simulink library "Cylinder_Lib"  (R2025a)
settings: Solver=ode45  StartTime=0.0  StopTime=10.0  RelTol=1e-3  EnableMultiTasking=on
undefined symbols (not defined in the file or in its folder): actuator_hs_b, actuator_hs_k
libraries: fl_lib x9, SimscapeFluids_lib x1
Description:
  | Copyright 2015-2025 The MathWorks, Inc.
settings Model: Creator=smiller  LastModifiedBy=smiller
settings SolverCC: AlgebraicLoopSolver=TrustRegion
settings DataIOCC: LimitDataPoints=on  SaveFormat=Array  ReturnWorkspaceOutputs=off
settings OptimizationCC: ReuseModelBlockBuffer=off  ExpressionDepthLimit=2147483647.0  LifeSpan=inf
settings DebuggingCC: UnderspecifiedInitializationDetection=Classic  MergeDetectMultiDrivingBlocksExec=none  SolverPrmCheckMsg=warning  UnconnectedInputMsg=warning  UnconnectedOutputMsg=warning  UnconnectedLineMsg=warning  AllowSymbolicDim=off  StateNameClashWarn=warning  PregeneratedLibrarySubsystemCodeDiagnostic=none  SFUnexpectedBacktrackingDiag=warning  SFNoUnconditionalDefaultTransitionDiag=warning  SFExecutionAtInitializationDiag=none  ArithmeticOperatorsInVariantConditions=warning
settings HardwareCC: ProdBitPerPointer=32.0  ProdBitPerSizeT=32.0  ProdBitPerPtrDiffT=32.0  ProdLargestAtomicFloat=None  ProdIntDivRoundTo=Undefined  ProdEndianess=Unspecified  ProdWordSize=32.0  ProdHWDeviceType=32-bit Generic
settings ModelReferenceCC: EnableRefExpFcnMdlSchedulingChecks=on  PropagateSignalLabelsOutOfModel=off
settings SFSimCC: SimUseLocalCustomCode=off  CustomCodeUndefinedFunction=UseInterfaceOnly
settings RTWCC: RTWUseLocalCustomCode=off  GPUComputeCapability=3.5  DLArmComputeVersion=19.05
settings CodeAppCC: StateflowObjectComments=on
settings GRTTargetCC: TargetLangStandard=C89/C90 (ANSI)
settings ConfigComp: CovMetricSettings=dw  CovSaveCumulativeToWorkspaceVar=on  CovSaveSingleToWorkspaceVar=on  CovExternalEMLEnable=off  CovSFcnEnable=off

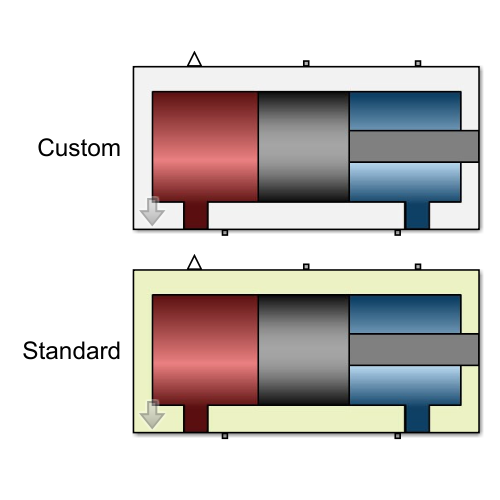
[thumbnail: Simulink's stored preview of the top-level diagram]
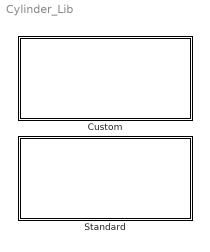
== system Cylinder_Lib ==
  Custom : Subsystem  VariantControl=Custom  mask(Double-Acting Hydraulic Actuator){A=5e-4, V=10e-5, PA=200, PB=0, T=200, hs_k=actuator_hs_k, hs_b=actuator_hs_b}
      mask prompts: A "Piston area (m^2)"; V "Chamber dead volume (m^3)"; PA "Chamber A initial pressure (bar)"; PB "Chamber B initial pressure (bar)"; T "Piston travel (mm)"; hs_k "Hardstop stiffness (N/m)"; hs_b "Hardstop damping (N/(m/s))"
      mask help: Models a double-acting hydraulic actuator using Simscape Foundation library components.
      mask Display: image('Double_Acting_Cylinder_Custom_IMAGE.jpg');
  Standard : Subsystem  VariantControl=Standard  mask(Double-Acting Hydraulic Actuator){A=5e-4, V=10e-5, PA=200, PB=0, T=200, hs_k=actuator_hs_k, hs_b=actuator_hs_b}
      mask prompts: A "Piston area (m^2)"; V "Chamber dead volume (m^3)"; PA "Chamber A initial pressure (bar)"; PB "Chamber B initial pressure (bar)"; T "Piston travel (mm)"; hs_k "Hardstop stiffness (N/m)"; hs_b "Hardstop damping (N/(m/s))"
      mask help: Models a double-acting hydraulic actuator using Simscape add-on library components.
      mask Display: image('Double_Acting_Cylinder_Standard_IMAGE.jpg');

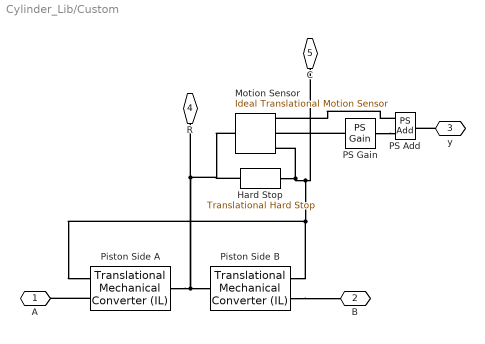
== system Cylinder_Lib/Custom ==
  " Motion Sensor" : fl_lib/Mechanical/Mechanical Sensors/Ideal Translational Motion Sensor  reference=foundation.enum.MeasurementReference.difference  acceleration_port=false  velocity_port=true  position_port=true  offset=Scissor_Lift_Param.Initial_Cyl_Ext mm
  Hard Stop : fl_lib/Mechanical/Translational Elements/Translational Hard Stop  upper_bnd=T/2 mm  lower_bnd=-T/2 mm  model=3  stiff_up=hs_k N/m  stiff_low=hs_k N/m  D_up=hs_b N/(m/s)  D_low=hs_b N/(m/s)  transition=0.1 mm  coeff_rest=0.7  v_tol=0.001 m/s  f_tol=0.001 N  v_specify=off  v_priority=High  v=0 m/s  v_nominal_specify=off  v_nominal_value=1  v_nominal_unit=m/s  f_specify=off  f_priority=High  f=0 N  f_nominal_specify=off  f_nominal_value=1  f_nominal_unit=N  x_specify=on  x_priority=High  x=0 m  x_nominal_specify=off  x_nominal_value=1  x_nominal_unit=m  M_specify=off  M_priority=None  M=0
  PS Add : fl_lib/Physical Signals/Functions/PS Add
  PS Gain : fl_lib/Physical Signals/Functions/PS Gain  gain=0.1 s
  Piston Side A : fl_lib/Isothermal Liquid/Elements/Translational Mechanical Converter (IL)  mech_orientation=1  displacement_spec=foundation.enum.DisplacementSpec.Calculate  x0=0 m  interface_area=A m^2  dead_volume=V m^3  pressure_spec=1  environment_pressure=0.101325 MPa  dynamic_compressibility=true  p0=0 + 101325 Pa  p_nominal=0.101325 MPa
      settings: LibrarySourceBlock=fl_lib/Isothermal Liquid/Elements/Translational Mechanical Converter (IL)  InternalSimscapePortConfiguration="{\"Bottom\":[],\"Left\":[{\"id\":\"A\",\"label\":\"A\",\"type\":\"foundation.isothermal_liquid.isothermal_liquid\"},{\"id\":\"C\",\"label\":\"C\",\"type\":\"foundation.mechanical.translational.translational\"}],\"Right\":[{\"id\":\"R\",\"label\":\"R\",\"type\":\"foundation.mechanical.translational.translational\"}],\"Top\":[]}"
  Piston Side B : fl_lib/Isothermal Liquid/Elements/Translational Mechanical Converter (IL)  mech_orientation=-1  displacement_spec=foundation.enum.DisplacementSpec.Calculate  x0=-(0) m  interface_area=A m^2  dead_volume=V m^3  pressure_spec=1  environment_pressure=0.101325 MPa  dynamic_compressibility=true  p0=0 + 101325 Pa  p_nominal=0.101325 MPa
      settings: LibrarySourceBlock=fl_lib/Isothermal Liquid/Elements/Translational Mechanical Converter (IL)  InternalSimscapePortConfiguration="{\"Bottom\":[],\"Left\":[{\"id\":\"A\",\"label\":\"A\",\"type\":\"foundation.isothermal_liquid.isothermal_liquid\"},{\"id\":\"C\",\"label\":\"C\",\"type\":\"foundation.mechanical.translational.translational\"}],\"Right\":[{\"id\":\"R\",\"label\":\"R\",\"type\":\"foundation.mechanical.translational.translational\"}],\"Top\":[]}"
  A : PMIOPort  Side=Left
  B : PMIOPort  Port=2  Side=Left
  y : PMIOPort  Port=3  Side=Right
  R : PMIOPort  Port=4  Side=Right
  C : PMIOPort  Port=5  Side=Right
  connections:
  PS Add/LConn1 -- " Motion Sensor"/RConn3
  Hard Stop/RConn1 -- Piston Side A/LConn2 -- Piston Side B/LConn2 -- C/RConn1 -- " Motion Sensor"/RConn1
  Piston Side A/LConn1 -- A/RConn1
  Piston Side B/LConn1 -- B/RConn1
  PS Gain/LConn1 -- " Motion Sensor"/RConn2
  y/RConn1 -- PS Add/RConn1
  PS Gain/RConn1 -- PS Add/LConn2
  Piston Side A/RConn1 -- Piston Side B/RConn1 -- R/RConn1 -- Hard Stop/LConn1 -- " Motion Sensor"/LConn1

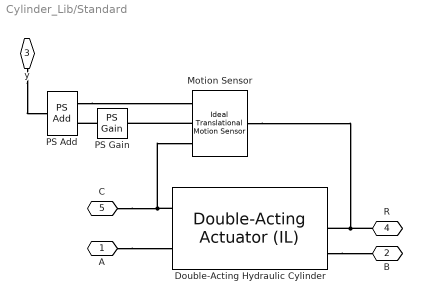
== system Cylinder_Lib/Standard ==
  " Motion Sensor" : fl_lib/Mechanical/Mechanical Sensors/Ideal Translational Motion Sensor  reference=foundation.enum.MeasurementReference.difference  acceleration_port=false  velocity_port=true  position_port=true  offset=Scissor_Lift_Param.Initial_Cyl_Ext mm
  Double-Acting Hydraulic Cylinder : SimscapeFluids_lib/Isothermal Liquid/Actuators/Double-Acting Actuator (IL)  single_fluid=true  mech_orientation=1  piston_area_A=A m^2  piston_area_B=A m^2  stroke=T mm  dead_volume_A=V m^3  dead_volume_B=V m^3  pressure_spec=foundation.enum.pressure_spec.atmospheric  environment_pressure=0.101325 MPa  hardstop_model=3  stiff_coeff=hs_k N/m  damping_coeff=hs_b N/(m/s)  transition=0.1 mm  coeff_rest=0.7  v_tol=0.001 m/s  f_tol=0.001 N  cushion_A_spec=false  area_plunger_A=1e-4 m^2  length_plunger_A=1e-3 m  area_cushion_orifice_A=1e-6 m^2  area_leak_plunger_A=1e-7 m^2  p_crack_differential_A=0.01 MPa  press_max_differential_A=0.1 MPa  check_valve_area_max_A=1e-4 m^2  check_valve_area_leak_A=1e-10 m^2  smoothing_factor_A=0  cushion_B_spec=false  area_plunger_B=1e-4 m^2  length_plunger_B=1e-3 m  area_cushion_orifice_B=1e-6 m^2  area_leak_plunger_B=1e-7 m^2  p_crack_differential_B=0.01 MPa  press_max_differential_B=0.1 MPa  check_valve_area_max_B=1e-4 m^2  check_valve_area_leak_B=1e-10 m^2  smoothing_factor_B=0  friction_spec=false  breakaway_Coulomb_ratio=1.2  breakaway_velocity=0.1 m/s  preload_force=20 N  Coulomb_coeff=1e-6 N/Pa  viscous_coeff=100 N*s/m  leakage_spec=false  clearance=1e-4 m  piston_length=0.01 m  displacement_spec=foundation.enum.DisplacementSpec.Calculate  x0=T/2 mm  dynamic_compressibility=true  p0_A=PA + 1.01325 bar  p0_B=PB + 1.01325 bar  p_nominal_A=0.101325 MPa  p_nominal_B=0.101325 MPa
      settings: LibrarySourceBlock=SimscapeFluids_lib/Isothermal Liquid/Actuators/Double-Acting Actuator (IL)  InternalSimscapePortConfiguration="{\"Bottom\":[],\"Left\":[{\"id\":\"C\",\"label\":\"C\",\"type\":\"foundation.mechanical.translational.translational\"},{\"id\":\"A\",\"label\":\"A\",\"type\":\"foundation.isothermal_liquid.isothermal_liquid\"}],\"Right\":[{\"id\":\"p_out\",\"label\":\"p\",\"type\":\"output\"},{\"id\":\"R\",\"label\":\"R\",\"type\":\"foundation.mechanical.translational.translational\"},{\"id\":\"B\",\"label\":\"B\",\"type\":\"foundation.isothermal_liquid.isothermal_liquid\"}],\"Top\":[]}"
  PS Add : fl_lib/Physical Signals/Functions/PS Add
  PS Gain : fl_lib/Physical Signals/Functions/PS Gain  gain=0.1 s
  A : PMIOPort  Side=Left
  B : PMIOPort  Port=2  Side=Left
  y : PMIOPort  Port=3  Side=Right
  R : PMIOPort  Port=4  Side=Right
  C : PMIOPort  Port=5  Side=Right
  connections:
  y/RConn1 -- PS Add/RConn1
  C/RConn1 -- Double-Acting Hydraulic Cylinder/LConn1 -- " Motion Sensor"/RConn1
  Double-Acting Hydraulic Cylinder/RConn3 -- B/RConn1
  PS Gain/RConn1 -- PS Add/LConn2
  " Motion Sensor"/RConn2 -- PS Gain/LConn1
  PS Add/LConn1 -- " Motion Sensor"/RConn3
  " Motion Sensor"/LConn1 -- R/RConn1 -- Double-Acting Hydraulic Cylinder/RConn2
  A/RConn1 -- Double-Acting Hydraulic Cylinder/LConn2
